simulink model "gfm_datacenter"  (R2018b)
settings: Solver=ode45  StartTime=0.0  StopTime=100  RelTol=1e-3
PreLoadFcn:
  | modelDir = fileparts(get_param(bdroot,'FileName'));
  | 
  | load_system(fullfile(modelDir,'controls_element_lib.slx'));
  | load_system(fullfile(modelDir,'test_sequence_lib.slx'));
InitFcn:
  | close all;
  | clear all;
  | clc;
  | 
  | close all;
  | clear all;
  | clc;
  | 
  | % frequency nominals
  | F_NOM = 60;
  | W_NOM = 2 * pi * F_NOM;
  | 
  | % base values relative to inverter
  | % --------------------------------
  | VLL_INV_NOM = 34.5e3;
  | P_INV_NOM = 5e6;
  | Q_INV_NOM = 2.5e6;
  | S_INV_NOM = sqrt(P_INV_NOM^2 + Q_INV_NOM^2);
  | 
  | I_INV_BASE = S_INV_NOM/(sqrt(3)*VLL_INV_NOM);
  | Z_INV_BASE = VLL_INV_NOM^2/S_INV_NOM;
  | L_INV_BASE = Z_INV_BASE / W_NOM;
  | C_INV_BASE = 1 / (Z_INV_BASE * W_NOM);
  | 
  | % SST Parameters
  | N_DCDC_XFMR = 3;
  | N_CELLS_PER_STRING = 10;
  | C_MV_CELL = 400e-6;
  | C_LV_SST = 5e-3;
  | C_BBU = 1500; % 60 sec * 5MW
  | r_BBU = 5e-3;
  | ILV_MAX = 300;
  | ILV_MIN = -300;
  | IMV_MAX = 100;
  | IMV_MIN = -100;
  | V_LVDC_NOM = 800;
  | IDC_NOM = P_INV_NOM / V_LVDC_NOM;
  | 
  | % nominal ratings for power system model
  | % --------------------------------------
  | INVERTER_COUNT = 20;
  | 
  | VMV_NOM = VLL_INV_NOM;
  | VHV_NOM = 230e3;
  | S_PLANT = INVERTER_COUNT * S_INV_NOM;
  | 
  | N_GSU = VHV_NOM/VMV_NOM;
  | 
  | I_MV_BASE = S_PLANT/(sqrt(3)*VMV_NOM);
  | I_HV_BASE = S_PLANT/(sqrt(3)*VHV_NOM);
  | 
  | Z_MV_BASE = VMV_NOM^2/S_PLANT;
  | Z_HV_BASE = VHV_NOM^2/S_PLANT;
  | 
  | L_MV_BASE = Z_MV_BASE / W_NOM;
  | L_HV_BASE = Z_HV_BASE / W_NOM;
  | C_MV_BASE = 1 / (Z_MV_BASE * W_NOM);
  | C_HV_BASE = 1 / (Z_HV_BASE * W_NOM);
libraries: test_sequence_lib x14, controls_element_lib x10
settings Model: SimulationMode=accelerator  Creator=halatrash  LastModifiedBy=ahhei
settings SolverCC: ZeroCrossAlgorithm=Adaptive
settings DataIOCC: ReturnWorkspaceOutputs=on
settings DebuggingCC: MaxConsecutiveZCsMsg=warning  IgnoredZcDiagnostic=none  UnconnectedInputMsg=none  UnconnectedOutputMsg=none  UnconnectedLineMsg=none
settings ModelReferenceCC: EnableRefExpFcnMdlSchedulingChecks=off
settings RTWCC: Description=Generic Real-Time Target
settings ConfigComp: CovBoundaryAbsTol=1.0e-5

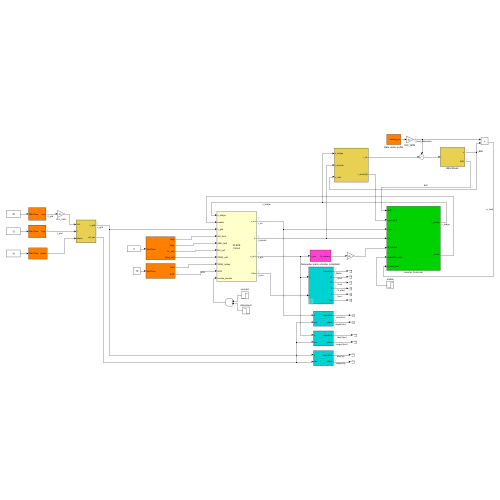
[thumbnail: Simulink's stored preview of the top-level diagram]
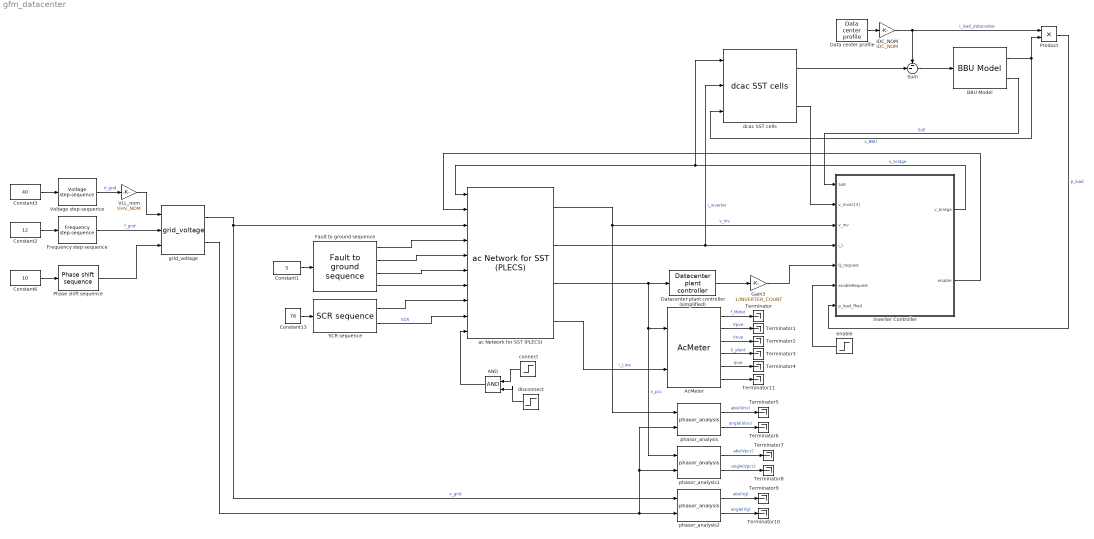
== system gfm_datacenter ==
  AND : Logic  IconShape=distinctive  AllPortsSameDT=off  OutDataTypeStr=boolean
  AcMeter : test_sequence_lib/AcMeter  VllRated=VHV_NOM
  BBU Model : test_sequence_lib/BBU Model  SystemSampleTime=-1  EmptyChoice=off  PassThrough=off  PassThroughVariantControl=(default)  EmptyChoiceVariantControl=(default)  Latency=0  AutoFrameSizeCalculation=off
  Constant1 : Constant  Value=5
  Constant13 : Constant  Value=78
  Constant2 : Constant  Value=12
  Constant3 : Constant  Value=40
  Constant6 : Constant  Value=10
  Data center profile : test_sequence_lib/Data center profile  SystemSampleTime=-1  EmptyChoice=off  PassThrough=off  PassThroughVariantControl=(default)  EmptyChoiceVariantControl=(default)  Latency=0  AutoFrameSizeCalculation=off
  Datacenter plant controller (simplified) : controls_element_lib/Datacenter plant controller  SystemSampleTime=-1  EmptyChoice=off  PassThrough=off  PassThroughVariantControl=(default)  EmptyChoiceVariantControl=(default)  Latency=0  AutoFrameSizeCalculation=off
  Fault to ground sequence : test_sequence_lib/Fault to ground sequence  SystemSampleTime=-1  EmptyChoice=off  PassThrough=off  PassThroughVariantControl=(default)  EmptyChoiceVariantControl=(default)  Latency=0  AutoFrameSizeCalculation=off
  Frequency step-sequence : test_sequence_lib/Frequency step-sequence  SystemSampleTime=-1  EmptyChoice=off  PassThrough=off  PassThroughVariantControl=(default)  EmptyChoiceVariantControl=(default)  Latency=0  AutoFrameSizeCalculation=off
  Gain3 : Gain  Gain=1/INVERTER_COUNT
  IDC_NOM : Gain  Gain=IDC_NOM
  Inverter Controller : Subsystem
  Phase shift sequence : test_sequence_lib/Phase shift sequence  SystemSampleTime=-1  EmptyChoice=off  PassThrough=off  PassThroughVariantControl=(default)  EmptyChoiceVariantControl=(default)  Latency=0  AutoFrameSizeCalculation=off
  Product : Product
  SCR sequence : test_sequence_lib/SCR sequence  SystemSampleTime=-1  EmptyChoice=off  PassThrough=off  PassThroughVariantControl=(default)  EmptyChoiceVariantControl=(default)  Latency=0  AutoFrameSizeCalculation=off
  Sum : Sum  Inputs=--|
  Terminator{,1..11} (12 alike) : Terminator
  VLL_nom : Gain  Gain=VHV_NOM
  Voltage step-sequence : test_sequence_lib/Voltage step-sequence  SystemSampleTime=-1  EmptyChoice=off  PassThrough=off  PassThroughVariantControl=(default)  EmptyChoiceVariantControl=(default)  Latency=0  AutoFrameSizeCalculation=off
  ac Network for SST (PLECS) : test_sequence_lib/ac Network for SST (PLECS)  PLECSData=<binary blob, 8352 chars, not shown>
  connect : Step  Time=0  SampleTime=0
  dcac SST cells : test_sequence_lib/dcac SST cells  SystemSampleTime=-1  EmptyChoice=off  PassThrough=off  PassThroughVariantControl=(default)  EmptyChoiceVariantControl=(default)  Latency=0  AutoFrameSizeCalculation=off
  disconnect : Step  Time=97  Before=1  After=0  SampleTime=0
  enable : Step  Time=2  SampleTime=0
  grid_voltage : test_sequence_lib/grid_voltage  SystemSampleTime=-1  EmptyChoice=off  PassThrough=off  PassThroughVariantControl=(default)  EmptyChoiceVariantControl=(default)  Latency=0  AutoFrameSizeCalculation=off
  phasor_analysis : test_sequence_lib/phasor_analysis  SystemSampleTime=-1  EmptyChoice=off  PassThrough=off  PassThroughVariantControl=(default)  EmptyChoiceVariantControl=(default)  Latency=0  AutoFrameSizeCalculation=off
  phasor_analysis1 : test_sequence_lib/phasor_analysis  SystemSampleTime=-1  EmptyChoice=off  PassThrough=off  PassThroughVariantControl=(default)  EmptyChoiceVariantControl=(default)  Latency=0  AutoFrameSizeCalculation=off
  phasor_analysis2 : test_sequence_lib/phasor_analysis  SystemSampleTime=-1  EmptyChoice=off  PassThrough=off  PassThroughVariantControl=(default)  EmptyChoiceVariantControl=(default)  Latency=0  AutoFrameSizeCalculation=off
  wires:
  enable/1 -> Inverter Controller/6(enableRequest)
  IDC_NOM/1 -> Sum/1, Product/1  "I_load_datacenter"
  Data center profile/1 -> IDC_NOM/1
  SCR sequence/2 -> ac Network for SST (PLECS)/9  "SCR"
  Inverter Controller/2(enable) -> ac Network for SST (PLECS)/2
  Constant1/1 -> Fault to ground sequence/1
  ac Network for SST (PLECS)/2 -> dcac SST cells/2, Inverter Controller/4(i_L)  "i_inverter"
  Frequency step-sequence/1 -> grid_voltage/2  "f_grid"
  Inverter Controller/1(v_bridge) -> dcac SST cells/1, ac Network for SST (PLECS)/1  "v_bridge"
  phasor_analysis/2 -> Terminator6/1  "angle(Vinv)"
  Fault to ground sequence/2 -> ac Network for SST (PLECS)/5
  AcMeter/3 -> Terminator2/1  "Vnve"
  ac Network for SST (PLECS)/3 -> Datacenter plant controller (simplified)/1, phasor_analysis1/1, AcMeter/1  "v_pcc"
  AcMeter/1 -> Terminator/1  "f_Meter"
  Gain3/1 -> Inverter Controller/5(Q_request)
  AcMeter/6 -> Terminator11/1
  grid_voltage/1 -> ac Network for SST (PLECS)/3, phasor_analysis2/1  "v_grid"
  Voltage step-sequence/1 -> VLL_nom/1  "V_grid"
  ac Network for SST (PLECS)/4 -> AcMeter/2  "i_Line"
  Constant6/1 -> Phase shift sequence/1
  Fault to ground sequence/4 -> ac Network for SST (PLECS)/7
  AcMeter/4 -> Terminator3/1  "S_plant"
  Constant3/1 -> Voltage step-sequence/1
  SCR sequence/1 -> ac Network for SST (PLECS)/8
  Constant2/1 -> Frequency step-sequence/1
  AcMeter/5 -> Terminator4/1  "Ipve"
  ac Network for SST (PLECS)/1 -> phasor_analysis/1, Inverter Controller/3(v_inv)  "v_inv"
  Phase shift sequence/1 -> grid_voltage/3
  Fault to ground sequence/3 -> ac Network for SST (PLECS)/6
  Fault to ground sequence/1 -> ac Network for SST (PLECS)/4
  Constant13/1 -> SCR sequence/1
  Datacenter plant controller (simplified)/1 -> Gain3/1
  phasor_analysis2/2 -> Terminator10/1  "angle(Vg)"
  disconnect/1 -> AND/2
  AcMeter/2 -> Terminator1/1  "Vpve"
  VLL_nom/1 -> grid_voltage/1
  phasor_analysis/1 -> Terminator5/1  "abs(Vinv)"
  phasor_analysis2/1 -> Terminator9/1  "abs(Vg)"
  AND/1 -> ac Network for SST (PLECS)/10
  connect/1 -> AND/1
  phasor_analysis1/1 -> Terminator7/1  "abs(Vpcc)"
  grid_voltage/2 -> phasor_analysis1/2, phasor_analysis/2, phasor_analysis2/2
  phasor_analysis1/2 -> Terminator8/1  "angle(Vpcc)"
  Sum/1 -> BBU Model/1
  BBU Model/1 -> dcac SST cells/3, Product/2  "v_BBU"
  Product/1 -> Inverter Controller/7(p_load_ffwd)  "p_load"
  dcac SST cells/1 -> Sum/2
  dcac SST cells/2 -> Inverter Controller/2(v_mvdc[3])
  BBU Model/2 -> Inverter Controller/1(SoE)  "SoE"

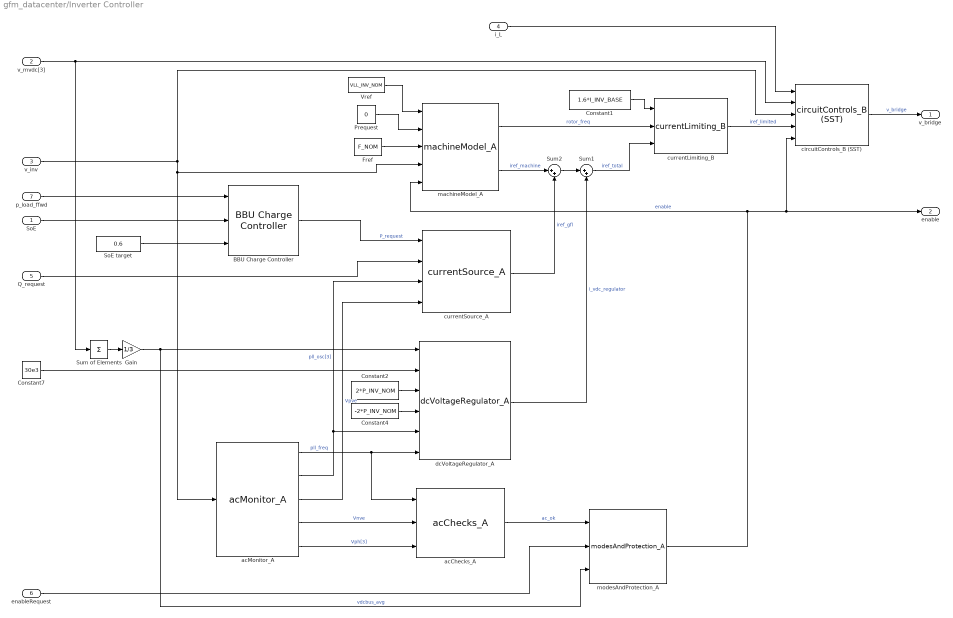
== system gfm_datacenter/Inverter Controller ==
  SoE : Inport
  v_mvdc[3] : Inport  Port=2
  v_inv : Inport  Port=3
  i_L : Inport  Port=4
  Q_request : Inport  Port=5
  enableRequest : Inport  Port=6
  p_load_ffwd : Inport  Port=7
  BBU Charge Controller : controls_element_lib/BBU Charge Controller  SystemSampleTime=-1  EmptyChoice=off  PassThrough=off  PassThroughVariantControl=(default)  EmptyChoiceVariantControl=(default)  Latency=0  AutoFrameSizeCalculation=off
  Constant1 : Constant  Value=1.6*I_INV_BASE
  Constant2 : Constant  Value=2*P_INV_NOM
  Constant4 : Constant  Value=-2*P_INV_NOM
  Constant7 : Constant  Value=30e3
  Fref : Constant  Value=F_NOM
  Gain : Gain  Gain=1/3
  Prequest : Constant  Value=0
  SoE target : Constant  Value=0.6
  Sum of Elements : Sum  Inputs=+
  Sum1 : Sum  Inputs=|++
  Sum2 : Sum  Inputs=|++
  Vref : Constant  Value=VLL_INV_NOM
  acChecks_A : controls_element_lib/acChecks_A  VllRated=VLL_INV_NOM  nominalFrequency=F_NOM  tRequalify=2  T_CNTL=1e-3
  acMonitor_A : controls_element_lib/acMonitor_A  VllRated=VLL_INV_NOM  nominalFrequency=F_NOM
  circuitControls_B (SST) : controls_element_lib/circuitControls_B (SST)  SystemSampleTime=-1  EmptyChoice=off  PassThrough=off  PassThroughVariantControl=(default)  EmptyChoiceVariantControl=(default)  Latency=0  AutoFrameSizeCalculation=off
  currentLimiting_B : controls_element_lib/currentLimiting_B  IRated=I_INV_BASE  peakSoftLimit=2.6  peakHardLimit=3.6
  currentSource_A : controls_element_lib/currentSource_A  VllRated=VLL_INV_NOM  SRated=S_INV_NOM  nominalFrequency=F_NOM  Plimit=P_INV_NOM/S_INV_NOM  Qlimit=Q_INV_NOM/S_INV_NOM
  dcVoltageRegulator_A : controls_element_lib/dcVoltageRegulator_A  kp=5e3  kSlowPath=0  wSlowPath=5  pLimitExternalMinimum=0.05*P_INV_NOM  vdc_deadband=1500  VllRated=VLL_INV_NOM
  machineModel_A : controls_element_lib/machineModel_A  SRated=S_INV_NOM  VllRated=VLL_INV_NOM  nominalFrequency=F_NOM  inertialConstant=2.5  kDroop=1  kDamper=2  Xs=0.3  rs=0.08  Qlimit=0.5  wExciter=10
  modesAndProtection_A : controls_element_lib/modesAndProtection_A  dcOvervotlageThreshold=40e3  dcUndervotlageThreshold=23e3  dcTripClearTimeout=0.2
  v_bridge : Outport
  enable : Outport  Port=2
  wires:
  Vref/1 -> machineModel_A/1
  Prequest/1 -> machineModel_A/2
  Fref/1 -> machineModel_A/3
  machineModel_A/2 -> Sum2/1  "iref_machine"
  currentLimiting_B/1 -> circuitControls_B (SST)/4  "iref_limited"
  v_inv/1 -> circuitControls_B (SST)/3, acMonitor_A/1, machineModel_A/4
  currentSource_A/1 -> Sum2/2  "iref_gfl"
  Sum1/1 -> currentLimiting_B/3  "iref_total"
  acMonitor_A/2 -> currentSource_A/3, dcVoltageRegulator_A/5  "pll_osc[3]"
  Q_request/1 -> currentSource_A/2
  acMonitor_A/4 -> acChecks_A/2  "Vnve"
  enableRequest/1 -> modesAndProtection_A/2
  modesAndProtection_A/1 -> machineModel_A/5, enable/1, circuitControls_B (SST)/5  "enable"
  BBU Charge Controller/1 -> currentSource_A/1  "P_request"
  acMonitor_A/3 -> currentSource_A/4  "Vpve"
  Constant1/1 -> currentLimiting_B/1
  acMonitor_A/5 -> acChecks_A/3  "Vph[3]"
  acChecks_A/1 -> modesAndProtection_A/1  "ac_ok"
  acMonitor_A/1 -> dcVoltageRegulator_A/6, acChecks_A/1  "pll_freq"
  dcVoltageRegulator_A/1 -> Sum1/2  "i_vdc_regulator"
  Sum2/1 -> Sum1/1
  Constant7/1 -> dcVoltageRegulator_A/2
  Sum of Elements/1 -> Gain/1
  Gain/1 -> modesAndProtection_A/3, dcVoltageRegulator_A/1  "vdcbus_avg"
  Constant2/1 -> dcVoltageRegulator_A/3
  Constant4/1 -> dcVoltageRegulator_A/4
  SoE/1 -> BBU Charge Controller/2
  p_load_ffwd/1 -> BBU Charge Controller/1
  circuitControls_B (SST)/1 -> v_bridge/1  "v_bridge"
  v_mvdc[3]/1 -> Sum of Elements/1, circuitControls_B (SST)/2
  i_L/1 -> circuitControls_B (SST)/1
  SoE target/1 -> BBU Charge Controller/3
  machineModel_A/1 -> currentLimiting_B/2  "rotor_freq"
